simulink model "r23_512p_fft"  (R2026b)
settings: Solver=FixedStepDiscrete  StopTime=5e-5*(127-1)  FixedStep=5e-5
libraries: dspsrcs4 x8
(part 3 of 3)

== matlab function r23_512p_fft/FFT_TOP/calc_unit11/bwr_unit ==
  data: si_cha input; so_cha output; so_chb output; si_chb input
function [so_cha, so_chb] = bwr_unit(si_cha, si_chb)
%BWR_UNIT Twiddle multiply after the butterfly: W^(3k), W^(7k), k = 0..63.

DW = 14;
LEN = 64;
KW  = 6;
fm = fimath('RoundingMethod', 'Nearest', 'OverflowAction', 'Saturate', ...
    'ProductMode', 'FullPrecision', 'SumMode', 'FullPrecision');
fc = fimath('RoundingMethod', 'Floor', 'OverflowAction', 'Wrap', ...
    'ProductMode', 'FullPrecision', 'SumMode', 'FullPrecision');
ROM_A_RE = coder.const(twiddle((0:LEN-1).' * 3, 1, fm));
ROM_A_IM = coder.const(twiddle((0:LEN-1).' * 3, 2, fm));
ROM_B_RE = coder.const(twiddle((0:LEN-1).' * 7, 1, fm));
ROM_B_IM = coder.const(twiddle((0:LEN-1).' * 7, 2, fm));

persistent k
if isempty(k)
    k = fi(LEN - 1, 0, KW, 0, fc);
end
if k == LEN - 1
    k(:) = 0;
else
    k(:) = k + 1;
end

so_cha = cmul(si_cha, [ROM_A_RE(k + 1), ROM_A_IM(k + 1)], DW, fm);
so_chb = cmul(si_chb, [ROM_B_RE(k + 1), ROM_B_IM(k + 1)], DW, fm);
end

function y = cmul(x, w, DW, fm)
y = fi(zeros(1, 2), 1, DW, 0, fm);
y(1) = x(1)*w(1) - x(2)*w(2);
y(2) = x(2)*w(1) + x(1)*w(2);
end

function w = twiddle(k, part, fm)
if part == 1
    w = fi(cos(2*pi*k/512), 1, 10, 8, fm);
else
    w = fi(-sin(2*pi*k/512), 1, 10, 8, fm);
end
end
